simulink model "battery"  (R2024a)
settings: Solver=ode23t  StartTime=0.0  StopTime=10000.0  MaxStep=5e-2  RelTol=1e-3
undefined symbols (not defined in the file or in its folder): battery_builder_rtmsupport, gcbh
libraries: fl_lib x8, batt_lib x8, nesl_utility x6, Batteries_thermal_lib x6, SimscapeFluids_lib x1, simulink x1
(part 2 of 2)

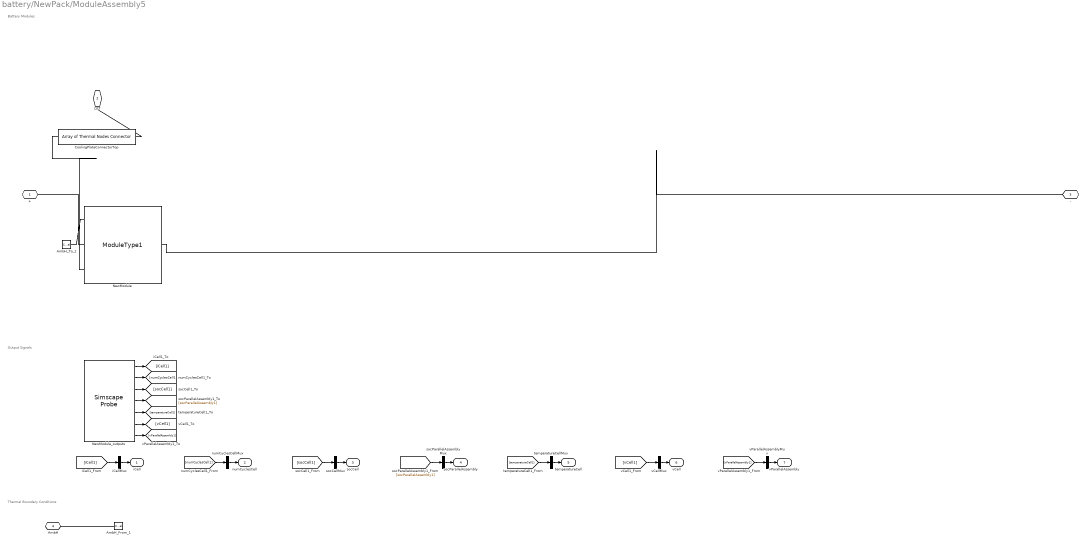
== system battery/NewPack/ModuleAssembly5 ==
  note: Thermal Boundary Conditions
  note: Output Signals
  note: Battery Modules
  AmbH_From_1 : ConnectionLabel  Label=ambH_1
  AmbH_To_1 : ConnectionLabel  Label=ambH_1
  CoolingPlateConnectorTop : batt_lib/Thermal/Array of Thermal Nodes Connector  numInputConnections=1  inNode1NumElements=1  inNode2NumElements=1  inNode3NumElements=1  inNode4NumElements=1  inNode5NumElements=1  inNode6NumElements=1  inNode7NumElements=1  inNode8NumElements=1  inNode9NumElements=1  inNode10NumElements=1  inNode11NumElements=1  inNode12NumElements=1  inNode13NumElements=1  inNode14NumElements=1  inNode15NumElements=1  inNode16NumElements=1  inNode17NumElements=1  inNode18NumElements=1  inNode19NumElements=1  inNode20NumElements=1  inNode21NumElements=1  inNode22NumElements=1  inNode23NumElements=1  inNode24NumElements=1  inNode25NumElements=1  inNode26NumElements=1  inNode27NumElements=1  inNode28NumElements=1  inNode29NumElements=1  inNode30NumElements=1  inNode31NumElements=1  inNode32NumElements=1  inNode33NumElements=1  inNode34NumElements=1  inNode35NumElements=1  inNode36NumElements=1  inNode37NumElements=1  inNode38NumElements=1  inNode39NumElements=1  inNode40NumElements=1  inNode41NumElements=1  inNode42NumElements=1  inNode43NumElements=1  inNode44NumElements=1  inNode45NumElements=1  inNode46NumElements=1  inNode47NumElements=1  inNode48NumElements=1  inNode49NumElements=1  inNode50NumElements=1
      settings: InternalSimscapePortConfiguration="{\"Bottom\":[{\"id\":\"outConn\",\"label\":\"outConn\",\"type\":\"foundation.thermal.thermal\"}],\"Left\":[],\"Right\":[],\"Top\":[{\"id\":\"inConn1\",\"label\":\"inConn1\",\"type\":\"foundation.thermal.thermal\"}]}"
  NewModule : Batteries_thermal_lib/Modules/ModuleType1  SOC_vecCell=[0, .1, .25, .5, .75, .9, 1]  T_vecCell=[278, 293, 313] K  V0_matCell=[3.49, 3.5, 3.51; 3.55, 3.57, 3.56; 3.62, 3.63, 3.64; 3.71, 3.71, 3.72; 3.91, 3.93, 3.94; 4.07, 4.08, 4.08; 4.19, 4.19, 4.19] V  V_rangeCell=[0, inf] V  R0_matCell=[.0117, .0085, .009; .011, .0085, .009; .0114, .0087, .0092; .0107, .0082, .0088; .0107, .0083, .0091; .0113, .0085, .0089; .0116, .0085, .0089] Ohm  AHCell=27 A*hr  extrapolation_optionCell=simscape.enum.extrapolation.nearest  thermal_massCell=100 J/K  CoolantResistance=1.2 K/W  AmbientResistance=25 K/W  P=1  S=1  iCell_specify=off  iCell_priority=None  iCell=0 A  iCell_nominal_specify=off  iCell_nominal_value=1  iCell_nominal_unit=A  vCell_specify=off  vCell_priority=None  vCell=0 V  vCell_nominal_specify=off  vCell_nominal_value=1  vCell_nominal_unit=V  socCell_specify=off  socCell_priority=High  socCell=1  socCell_nominal_specify=off  socCell_nominal_value=1  socCell_nominal_unit=1  numCyclesCell_specify=off  numCyclesCell_priority=High  numCyclesCell=0  numCyclesCell_nominal_specify=off  numCyclesCell_nominal_value=1  numCyclesCell_nominal_unit=1  temperatureCell_specify=off  temperatureCell_priority=High  temperatureCell=298.15 K  temperatureCell_nominal_specify=off  temperatureCell_nominal_value=1  temperatureCell_nominal_unit=K  vParallelAssembly_specify=off  vParallelAssembly_priority=None  vParallelAssembly=0 V  vParallelAssembly_nominal_specify=off  vParallelAssembly_nominal_value=1  vParallelAssembly_nominal_unit=V  socParallelAssembly_specify=off  socParallelAssembly_priority=None  socParallelAssembly=1  socParallelAssembly_nominal_specify=off  socParallelAssembly_nominal_value=1  socParallelAssembly_nominal_unit=1
      settings: InternalSimscapePortConfiguration="{\"Bottom\":[{\"id\":\"n\",\"label\":\"-\",\"type\":\"foundation.electrical.electrical\"}],\"Left\":[{\"id\":\"AmbH\",\"label\":\"AmbH\",\"type\":\"foundation.thermal.thermal\"}],\"Right\":[],\"Top\":[{\"id\":\"p\",\"label\":\"+\",\"type\":\"foundation.electrical.electrical\"},{\"id\":\"TopExtClnt\",\"label\":\"CPT\",\"type\":\"foundation.thermal.thermal\"}]}"
  NewModule_outputs : SimscapeProbe  BoundBlock=152  Variables={iCell, numCyclesCell, socCell, socParallelAssembly, temperatureCell, vCell, vParallelAssembly}
  iCellMux : Mux  Inputs=1
  numCyclesCellMux : Mux  Inputs=1
  socCellMux : Mux  Inputs=1
  socParallelAssemblyMux : Mux  Inputs=1
  temperatureCellMux : Mux  Inputs=1
  vCellMux : Mux  Inputs=1
  vParallelAssemblyMux : Mux  Inputs=1
  + : PMIOPort  Side=Left
  CPT : PMIOPort  Port=2  Side=Left  ConnectionType=Connection: foundation.thermal.thermal
  - : PMIOPort  Port=3  Side=Right
  AmbH : PMIOPort  Port=4  Side=Right  ConnectionType=Connection: foundation.thermal.thermal
  iCell : Outport
  numCyclesCell : Outport  Port=2
  socCell : Outport  Port=3
  socParallelAssembly : Outport  Port=4
  temperatureCell : Outport  Port=5
  vCell : Outport  Port=6
  vParallelAssembly : Outport  Port=7
  wires:
  [vParallelAssembly1] -> vParallelAssemblyMux/1
  vParallelAssemblyMux/1 -> vParallelAssembly/1
  NewModule_outputs/7 -> [vParallelAssembly1]
  [vCell1] -> vCellMux/1
  vCellMux/1 -> vCell/1
  NewModule_outputs/6 -> [vCell1]
  [temperatureCell1] -> temperatureCellMux/1
  temperatureCellMux/1 -> temperatureCell/1
  NewModule_outputs/5 -> [temperatureCell1]
  [socParallelAssembly1] -> socParallelAssemblyMux/1
  socParallelAssemblyMux/1 -> socParallelAssembly/1
  NewModule_outputs/4 -> [socParallelAssembly1]
  [socCell1] -> socCellMux/1
  socCellMux/1 -> socCell/1
  NewModule_outputs/3 -> [socCell1]
  [numCyclesCell1] -> numCyclesCellMux/1
  numCyclesCellMux/1 -> numCyclesCell/1
  NewModule_outputs/2 -> [numCyclesCell1]
  [iCell1] -> iCellMux/1
  iCellMux/1 -> iCell/1
  NewModule_outputs/1 -> [iCell1]
  connections:
  CoolingPlateConnectorTop/RConn1 -- CPT/RConn1
  CoolingPlateConnectorTop/LConn1 -- NewModule/LConn3
  AmbH_From_1/LConn1 -- AmbH/RConn1
  AmbH_To_1/LConn1 -- NewModule/LConn1
  NewModule/RConn1 -- -/RConn1
  NewModule/LConn2 -- +/RConn1

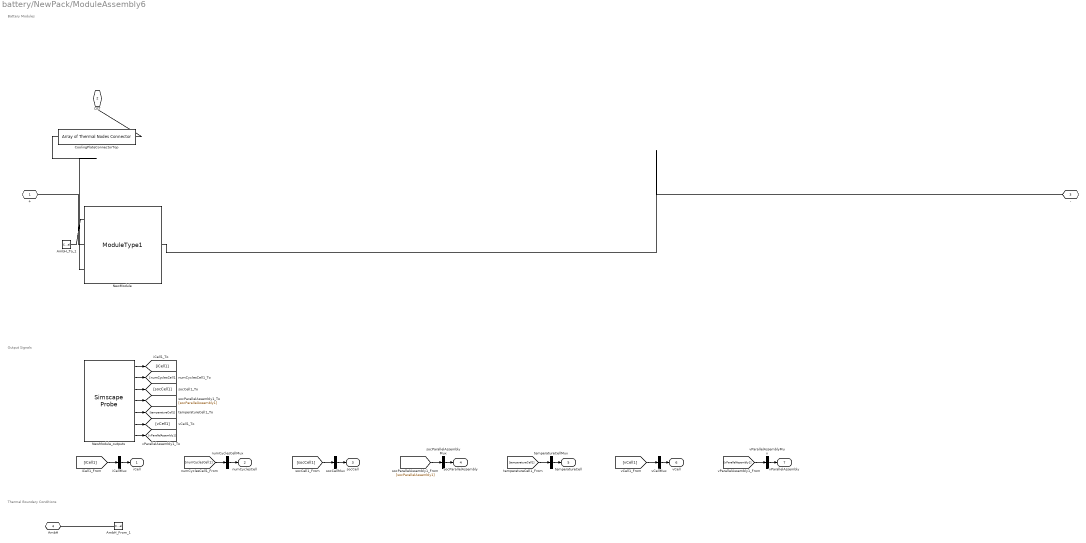
== system battery/NewPack/ModuleAssembly6 ==
  note: Thermal Boundary Conditions
  note: Output Signals
  note: Battery Modules
  AmbH_From_1 : ConnectionLabel  Label=ambH_1
  AmbH_To_1 : ConnectionLabel  Label=ambH_1
  CoolingPlateConnectorTop : batt_lib/Thermal/Array of Thermal Nodes Connector  numInputConnections=1  inNode1NumElements=1  inNode2NumElements=1  inNode3NumElements=1  inNode4NumElements=1  inNode5NumElements=1  inNode6NumElements=1  inNode7NumElements=1  inNode8NumElements=1  inNode9NumElements=1  inNode10NumElements=1  inNode11NumElements=1  inNode12NumElements=1  inNode13NumElements=1  inNode14NumElements=1  inNode15NumElements=1  inNode16NumElements=1  inNode17NumElements=1  inNode18NumElements=1  inNode19NumElements=1  inNode20NumElements=1  inNode21NumElements=1  inNode22NumElements=1  inNode23NumElements=1  inNode24NumElements=1  inNode25NumElements=1  inNode26NumElements=1  inNode27NumElements=1  inNode28NumElements=1  inNode29NumElements=1  inNode30NumElements=1  inNode31NumElements=1  inNode32NumElements=1  inNode33NumElements=1  inNode34NumElements=1  inNode35NumElements=1  inNode36NumElements=1  inNode37NumElements=1  inNode38NumElements=1  inNode39NumElements=1  inNode40NumElements=1  inNode41NumElements=1  inNode42NumElements=1  inNode43NumElements=1  inNode44NumElements=1  inNode45NumElements=1  inNode46NumElements=1  inNode47NumElements=1  inNode48NumElements=1  inNode49NumElements=1  inNode50NumElements=1
      settings: InternalSimscapePortConfiguration="{\"Bottom\":[{\"id\":\"outConn\",\"label\":\"outConn\",\"type\":\"foundation.thermal.thermal\"}],\"Left\":[],\"Right\":[],\"Top\":[{\"id\":\"inConn1\",\"label\":\"inConn1\",\"type\":\"foundation.thermal.thermal\"}]}"
  NewModule : Batteries_thermal_lib/Modules/ModuleType1  SOC_vecCell=[0, .1, .25, .5, .75, .9, 1]  T_vecCell=[278, 293, 313] K  V0_matCell=[3.49, 3.5, 3.51; 3.55, 3.57, 3.56; 3.62, 3.63, 3.64; 3.71, 3.71, 3.72; 3.91, 3.93, 3.94; 4.07, 4.08, 4.08; 4.19, 4.19, 4.19] V  V_rangeCell=[0, inf] V  R0_matCell=[.0117, .0085, .009; .011, .0085, .009; .0114, .0087, .0092; .0107, .0082, .0088; .0107, .0083, .0091; .0113, .0085, .0089; .0116, .0085, .0089] Ohm  AHCell=27 A*hr  extrapolation_optionCell=simscape.enum.extrapolation.nearest  thermal_massCell=100 J/K  CoolantResistance=1.2 K/W  AmbientResistance=25 K/W  P=1  S=1  iCell_specify=off  iCell_priority=None  iCell=0 A  iCell_nominal_specify=off  iCell_nominal_value=1  iCell_nominal_unit=A  vCell_specify=off  vCell_priority=None  vCell=0 V  vCell_nominal_specify=off  vCell_nominal_value=1  vCell_nominal_unit=V  socCell_specify=off  socCell_priority=High  socCell=1  socCell_nominal_specify=off  socCell_nominal_value=1  socCell_nominal_unit=1  numCyclesCell_specify=off  numCyclesCell_priority=High  numCyclesCell=0  numCyclesCell_nominal_specify=off  numCyclesCell_nominal_value=1  numCyclesCell_nominal_unit=1  temperatureCell_specify=off  temperatureCell_priority=High  temperatureCell=298.15 K  temperatureCell_nominal_specify=off  temperatureCell_nominal_value=1  temperatureCell_nominal_unit=K  vParallelAssembly_specify=off  vParallelAssembly_priority=None  vParallelAssembly=0 V  vParallelAssembly_nominal_specify=off  vParallelAssembly_nominal_value=1  vParallelAssembly_nominal_unit=V  socParallelAssembly_specify=off  socParallelAssembly_priority=None  socParallelAssembly=1  socParallelAssembly_nominal_specify=off  socParallelAssembly_nominal_value=1  socParallelAssembly_nominal_unit=1
      settings: InternalSimscapePortConfiguration="{\"Bottom\":[{\"id\":\"n\",\"label\":\"-\",\"type\":\"foundation.electrical.electrical\"}],\"Left\":[{\"id\":\"AmbH\",\"label\":\"AmbH\",\"type\":\"foundation.thermal.thermal\"}],\"Right\":[],\"Top\":[{\"id\":\"p\",\"label\":\"+\",\"type\":\"foundation.electrical.electrical\"},{\"id\":\"TopExtClnt\",\"label\":\"CPT\",\"type\":\"foundation.thermal.thermal\"}]}"
  NewModule_outputs : SimscapeProbe  BoundBlock=193  Variables={iCell, numCyclesCell, socCell, socParallelAssembly, temperatureCell, vCell, vParallelAssembly}
  iCellMux : Mux  Inputs=1
  numCyclesCellMux : Mux  Inputs=1
  socCellMux : Mux  Inputs=1
  socParallelAssemblyMux : Mux  Inputs=1
  temperatureCellMux : Mux  Inputs=1
  vCellMux : Mux  Inputs=1
  vParallelAssemblyMux : Mux  Inputs=1
  + : PMIOPort  Side=Left
  CPT : PMIOPort  Port=2  Side=Left  ConnectionType=Connection: foundation.thermal.thermal
  - : PMIOPort  Port=3  Side=Right
  AmbH : PMIOPort  Port=4  Side=Right  ConnectionType=Connection: foundation.thermal.thermal
  iCell : Outport
  numCyclesCell : Outport  Port=2
  socCell : Outport  Port=3
  socParallelAssembly : Outport  Port=4
  temperatureCell : Outport  Port=5
  vCell : Outport  Port=6
  vParallelAssembly : Outport  Port=7
  wires:
  [vParallelAssembly1] -> vParallelAssemblyMux/1
  vParallelAssemblyMux/1 -> vParallelAssembly/1
  NewModule_outputs/7 -> [vParallelAssembly1]
  [vCell1] -> vCellMux/1
  vCellMux/1 -> vCell/1
  NewModule_outputs/6 -> [vCell1]
  [temperatureCell1] -> temperatureCellMux/1
  temperatureCellMux/1 -> temperatureCell/1
  NewModule_outputs/5 -> [temperatureCell1]
  [socParallelAssembly1] -> socParallelAssemblyMux/1
  socParallelAssemblyMux/1 -> socParallelAssembly/1
  NewModule_outputs/4 -> [socParallelAssembly1]
  [socCell1] -> socCellMux/1
  socCellMux/1 -> socCell/1
  NewModule_outputs/3 -> [socCell1]
  [numCyclesCell1] -> numCyclesCellMux/1
  numCyclesCellMux/1 -> numCyclesCell/1
  NewModule_outputs/2 -> [numCyclesCell1]
  [iCell1] -> iCellMux/1
  iCellMux/1 -> iCell/1
  NewModule_outputs/1 -> [iCell1]
  connections:
  CoolingPlateConnectorTop/RConn1 -- CPT/RConn1
  CoolingPlateConnectorTop/LConn1 -- NewModule/LConn3
  AmbH_From_1/LConn1 -- AmbH/RConn1
  AmbH_To_1/LConn1 -- NewModule/LConn1
  NewModule/RConn1 -- -/RConn1
  NewModule/LConn2 -- +/RConn1

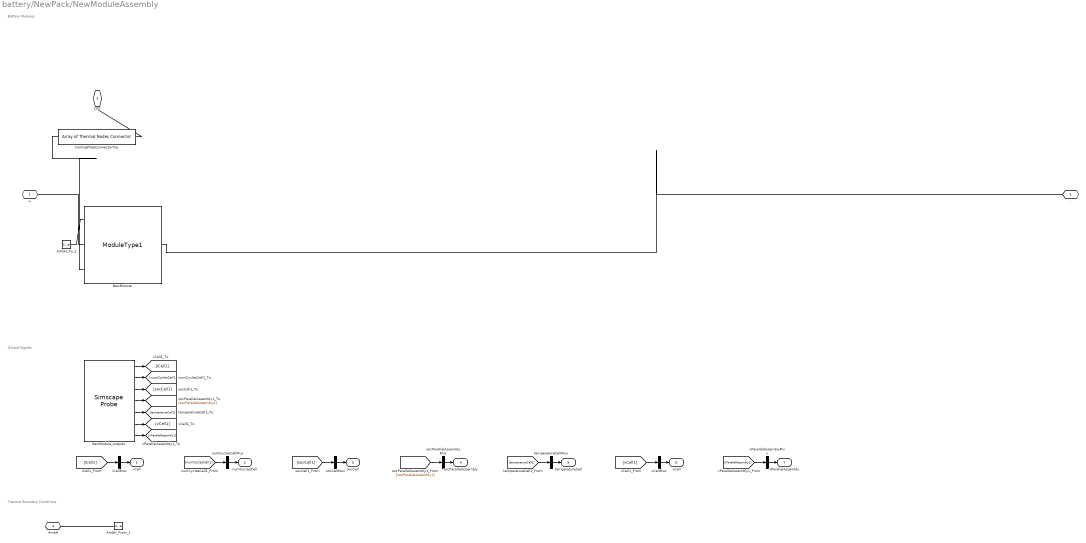
== system battery/NewPack/NewModuleAssembly ==
  note: Thermal Boundary Conditions
  note: Output Signals
  note: Battery Modules
  AmbH_From_1 : ConnectionLabel  Label=ambH_1
  AmbH_To_1 : ConnectionLabel  Label=ambH_1
  CoolingPlateConnectorTop : batt_lib/Thermal/Array of Thermal Nodes Connector  numInputConnections=1  inNode1NumElements=1  inNode2NumElements=1  inNode3NumElements=1  inNode4NumElements=1  inNode5NumElements=1  inNode6NumElements=1  inNode7NumElements=1  inNode8NumElements=1  inNode9NumElements=1  inNode10NumElements=1  inNode11NumElements=1  inNode12NumElements=1  inNode13NumElements=1  inNode14NumElements=1  inNode15NumElements=1  inNode16NumElements=1  inNode17NumElements=1  inNode18NumElements=1  inNode19NumElements=1  inNode20NumElements=1  inNode21NumElements=1  inNode22NumElements=1  inNode23NumElements=1  inNode24NumElements=1  inNode25NumElements=1  inNode26NumElements=1  inNode27NumElements=1  inNode28NumElements=1  inNode29NumElements=1  inNode30NumElements=1  inNode31NumElements=1  inNode32NumElements=1  inNode33NumElements=1  inNode34NumElements=1  inNode35NumElements=1  inNode36NumElements=1  inNode37NumElements=1  inNode38NumElements=1  inNode39NumElements=1  inNode40NumElements=1  inNode41NumElements=1  inNode42NumElements=1  inNode43NumElements=1  inNode44NumElements=1  inNode45NumElements=1  inNode46NumElements=1  inNode47NumElements=1  inNode48NumElements=1  inNode49NumElements=1  inNode50NumElements=1
      settings: InternalSimscapePortConfiguration="{\"Bottom\":[{\"id\":\"outConn\",\"label\":\"outConn\",\"type\":\"foundation.thermal.thermal\"}],\"Left\":[],\"Right\":[],\"Top\":[{\"id\":\"inConn1\",\"label\":\"inConn1\",\"type\":\"foundation.thermal.thermal\"}]}"
  NewModule : Batteries_thermal_lib/Modules/ModuleType1  SOC_vecCell=[0, .1, .25, .5, .75, .9, 1]  T_vecCell=[278, 293, 313] K  V0_matCell=[3.49, 3.5, 3.51; 3.55, 3.57, 3.56; 3.62, 3.63, 3.64; 3.71, 3.71, 3.72; 3.91, 3.93, 3.94; 4.07, 4.08, 4.08; 4.19, 4.19, 4.19] V  V_rangeCell=[0, inf] V  R0_matCell=[.0117, .0085, .009; .011, .0085, .009; .0114, .0087, .0092; .0107, .0082, .0088; .0107, .0083, .0091; .0113, .0085, .0089; .0116, .0085, .0089] Ohm  AHCell=27 A*hr  extrapolation_optionCell=simscape.enum.extrapolation.nearest  thermal_massCell=100 J/K  CoolantResistance=1.2 K/W  AmbientResistance=25 K/W  P=1  S=1  iCell_specify=off  iCell_priority=None  iCell=0 A  iCell_nominal_specify=off  iCell_nominal_value=1  iCell_nominal_unit=A  vCell_specify=off  vCell_priority=None  vCell=0 V  vCell_nominal_specify=off  vCell_nominal_value=1  vCell_nominal_unit=V  socCell_specify=off  socCell_priority=High  socCell=1  socCell_nominal_specify=off  socCell_nominal_value=1  socCell_nominal_unit=1  numCyclesCell_specify=off  numCyclesCell_priority=High  numCyclesCell=0  numCyclesCell_nominal_specify=off  numCyclesCell_nominal_value=1  numCyclesCell_nominal_unit=1  temperatureCell_specify=off  temperatureCell_priority=High  temperatureCell=298.15 K  temperatureCell_nominal_specify=off  temperatureCell_nominal_value=1  temperatureCell_nominal_unit=K  vParallelAssembly_specify=off  vParallelAssembly_priority=None  vParallelAssembly=0 V  vParallelAssembly_nominal_specify=off  vParallelAssembly_nominal_value=1  vParallelAssembly_nominal_unit=V  socParallelAssembly_specify=off  socParallelAssembly_priority=None  socParallelAssembly=1  socParallelAssembly_nominal_specify=off  socParallelAssembly_nominal_value=1  socParallelAssembly_nominal_unit=1
      settings: InternalSimscapePortConfiguration="{\"Bottom\":[{\"id\":\"n\",\"label\":\"-\",\"type\":\"foundation.electrical.electrical\"}],\"Left\":[{\"id\":\"AmbH\",\"label\":\"AmbH\",\"type\":\"foundation.thermal.thermal\"}],\"Right\":[],\"Top\":[{\"id\":\"p\",\"label\":\"+\",\"type\":\"foundation.electrical.electrical\"},{\"id\":\"TopExtClnt\",\"label\":\"CPT\",\"type\":\"foundation.thermal.thermal\"}]}"
  NewModule_outputs : SimscapeProbe  BoundBlock=235  Variables={iCell, numCyclesCell, socCell, socParallelAssembly, temperatureCell, vCell, vParallelAssembly}
  iCellMux : Mux  Inputs=1
  numCyclesCellMux : Mux  Inputs=1
  socCellMux : Mux  Inputs=1
  socParallelAssemblyMux : Mux  Inputs=1
  temperatureCellMux : Mux  Inputs=1
  vCellMux : Mux  Inputs=1
  vParallelAssemblyMux : Mux  Inputs=1
  + : PMIOPort  Side=Left
  CPT : PMIOPort  Port=2  Side=Left  ConnectionType=Connection: foundation.thermal.thermal
  - : PMIOPort  Port=3  Side=Right
  AmbH : PMIOPort  Port=4  Side=Right  ConnectionType=Connection: foundation.thermal.thermal
  iCell : Outport
  numCyclesCell : Outport  Port=2
  socCell : Outport  Port=3
  socParallelAssembly : Outport  Port=4
  temperatureCell : Outport  Port=5
  vCell : Outport  Port=6
  vParallelAssembly : Outport  Port=7
  wires:
  [vParallelAssembly1] -> vParallelAssemblyMux/1
  vParallelAssemblyMux/1 -> vParallelAssembly/1
  NewModule_outputs/7 -> [vParallelAssembly1]
  [vCell1] -> vCellMux/1
  vCellMux/1 -> vCell/1
  NewModule_outputs/6 -> [vCell1]
  [temperatureCell1] -> temperatureCellMux/1
  temperatureCellMux/1 -> temperatureCell/1
  NewModule_outputs/5 -> [temperatureCell1]
  [socParallelAssembly1] -> socParallelAssemblyMux/1
  socParallelAssemblyMux/1 -> socParallelAssembly/1
  NewModule_outputs/4 -> [socParallelAssembly1]
  [socCell1] -> socCellMux/1
  socCellMux/1 -> socCell/1
  NewModule_outputs/3 -> [socCell1]
  [numCyclesCell1] -> numCyclesCellMux/1
  numCyclesCellMux/1 -> numCyclesCell/1
  NewModule_outputs/2 -> [numCyclesCell1]
  [iCell1] -> iCellMux/1
  iCellMux/1 -> iCell/1
  NewModule_outputs/1 -> [iCell1]
  connections:
  CoolingPlateConnectorTop/RConn1 -- CPT/RConn1
  CoolingPlateConnectorTop/LConn1 -- NewModule/LConn3
  AmbH_From_1/LConn1 -- AmbH/RConn1
  AmbH_To_1/LConn1 -- NewModule/LConn1
  NewModule/RConn1 -- -/RConn1
  NewModule/LConn2 -- +/RConn1
